simulink model "threePhaseSinePWM"  (R2024b)
settings: Solver=VariableStepAuto  StartTime=0.0  StopTime=5  RelTol=1e-3
libraries: spsMosfetLib x6, spsThreePhaseSeriesRLCBranchLib x2, spsThreePhaseVIMeasurementLib x2, spsDCVoltageSourceLib x1, spsGroundLib x1, spsTriangleGeneratorLib x1, spspowerguiLib x1
settings Model: Creator=lenovo  LastModifiedBy=lenovo

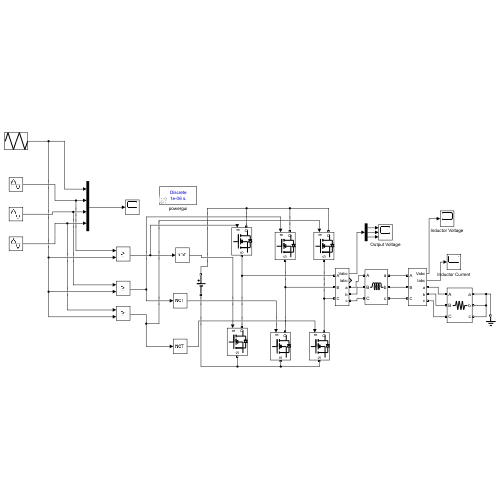
[thumbnail: Simulink's stored preview of the top-level diagram]
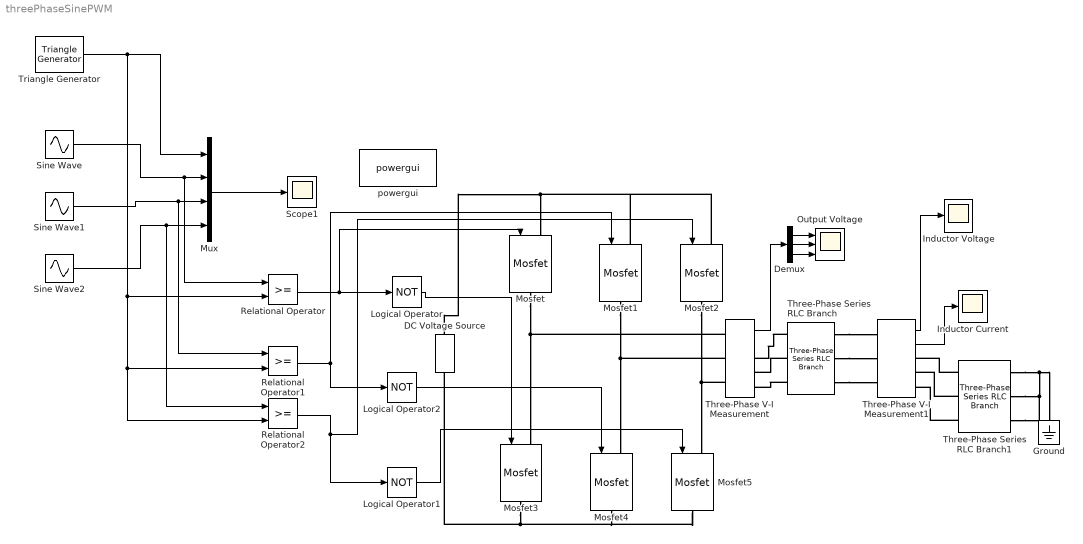
== system threePhaseSinePWM ==
  DC Voltage Source : spsDCVoltageSourceLib/DC Voltage Source  Amplitude=800  Measurements=None
  Demux : Demux  Outputs=3
  Ground : spsGroundLib/Ground  LConnTagsString=a
  Inductor Current : Scope
  Inductor Voltage : Scope
  Logical Operator : Logic  Operator=NOT  AllPortsSameDT=off  OutDataTypeStr=boolean
  Logical Operator1 : Logic  Operator=NOT  AllPortsSameDT=off  OutDataTypeStr=boolean
  Logical Operator2 : Logic  Operator=NOT  AllPortsSameDT=off  OutDataTypeStr=boolean
  Mosfet{,1..5} (6 alike) : spsMosfetLib/Mosfet  Ron=0.1  Lon=0  Rd=0.01  Vfd=0  IC=0  Rs=1e5  Cs=inf  Measurements=off
  Mux : Mux
  Output Voltage : Scope  NumInputPorts=3
  Relational Operator : RelationalOperator  OutDataTypeStr=boolean  RndMeth=Simplest  InputSameDT=off
  Relational Operator1 : RelationalOperator  OutDataTypeStr=boolean  RndMeth=Simplest  InputSameDT=off
  Relational Operator2 : RelationalOperator  OutDataTypeStr=boolean  RndMeth=Simplest  InputSameDT=off
  Scope1 : Scope
  Sine Wave : Sin  Amplitude=0.8  Frequency=2*pi*50  SampleTime=0
  Sine Wave1 : Sin  Amplitude=0.8  Frequency=2*pi*50  Phase=2*pi*50/3  SampleTime=0
  Sine Wave2 : Sin  Amplitude=0.8  Frequency=2*pi*50  Phase=-2*pi*50/3  SampleTime=0
  Three-Phase Series RLC Branch : spsThreePhaseSeriesRLCBranchLib/Three-Phase Series RLC Branch  LConnTagsString=A|B|C  RConnTagsString=A|B|C  BranchType=L  Resistance=1  Inductance=9e-3  Capacitance=1e-6  Measurements=None
  Three-Phase Series RLC Branch1 : spsThreePhaseSeriesRLCBranchLib/Three-Phase Series RLC Branch  LConnTagsString=A|B|C  RConnTagsString=A|B|C  BranchType=R  Resistance=5  Inductance=1e-3  Capacitance=1e-6  Measurements=None
  Three-Phase V-I Measurement : spsThreePhaseVIMeasurementLib/Three-Phase V-I Measurement  VoltageMeasurement=phase-to-ground  SetLabelV=off  LabelV=Vabc  Vpu=off  VpuLL=off  CurrentMeasurement=yes  SetLabelI=off  LabelI=Iabc  Ipu=off  Pbase=100e6  Vbase=500e3  OutputType=Complex  PhasorSimulation=off  PSBequivalent=0
  Three-Phase V-I Measurement1 : spsThreePhaseVIMeasurementLib/Three-Phase V-I Measurement  VoltageMeasurement=phase-to-ground  SetLabelV=off  LabelV=VabcL  Vpu=off  VpuLL=off  CurrentMeasurement=yes  SetLabelI=off  LabelI=IabcL  Ipu=off  Pbase=100e6  Vbase=500e3  OutputType=Complex  PhasorSimulation=off  PSBequivalent=0
  Triangle Generator : spsTriangleGeneratorLib/Triangle Generator  Freq=10e3  Phase=90  Ts=0
  powergui : spspowerguiLib/powergui  Priority=1  SimulationMode=Discrete  SampleTime=1e-6  frequency=60  Iterations=50  frequencyindice=0  Pbase=100e6  ErrMax=1e-4  UnitsV=kV  UnitsW=MW  buscounter=0  FunctionMessages=off  echomessages=off  EnableUseOfTLC=off  CurrentSourceSwitches=off  DisableSnubberDevices=off  DisableRonSwitches=off  DisableVfSwitches=off  DisplayEquations=off  AutomaticDiscreteSolvers=off  SolverType=Tustin/Backward Euler (TBE)  Interpol=off  ExternalGateDelay=off  methode=off  Ts=100  x0status=blocks  SPID=on  SwTol=0  HookPort=off  NonlinearTolerance=1e-4  nMaxIteration=100  ContinueOnMaxIteration=off  RestoreLinks=warning  ResistiveCurrentMeasurement=off  Frange=[0:2:500]  Ylog=off  Xlog=on  ShowGrid=off  save=off  variable=ZData  structure=0  ZoomFFT=off  StartTime=0.0  cycles=1  DisplayStyle=1  fundamental=60  FreqAxis=off  MaxFrequency=1000  frequencyindicesteady=1  RmsSteady=1  display=off
  wires:
  Mux/1 -> Scope1/1
  Sine Wave2/1 -> Mux/4, Relational Operator2/1
  Sine Wave1/1 -> Mux/3, Relational Operator1/1
  Sine Wave/1 -> Mux/2, Relational Operator/1
  Triangle Generator/1 -> Mux/1, Relational Operator2/2, Relational Operator1/2, Relational Operator/2
  Relational Operator/1 -> Mosfet/1, Logical Operator/1
  Logical Operator1/1 -> Mosfet5/1
  Logical Operator2/1 -> Mosfet4/1
  Logical Operator/1 -> Mosfet3/1
  Relational Operator1/1 -> Mosfet1/1, Logical Operator2/1
  Relational Operator2/1 -> Mosfet2/1, Logical Operator1/1
  Three-Phase V-I Measurement1/1 -> Inductor Voltage/1
  Three-Phase V-I Measurement1/2 -> Inductor Current/1
  Demux/3 -> Output Voltage/3
  Demux/1 -> Output Voltage/1
  Demux/2 -> Output Voltage/2
  Three-Phase V-I Measurement/1 -> Demux/1
  connections:
  Mosfet/RConn1 -- Mosfet3/LConn1 -- Three-Phase V-I Measurement/LConn1
  Mosfet1/RConn1 -- Mosfet4/LConn1 -- Three-Phase V-I Measurement/LConn2
  Mosfet2/RConn1 -- Mosfet5/LConn1 -- Three-Phase V-I Measurement/LConn3
  DC Voltage Source/RConn1 -- Mosfet2/LConn1 -- Mosfet1/LConn1 -- Mosfet/LConn1
  Mosfet3/RConn1 -- Mosfet5/RConn1 -- Mosfet4/RConn1 -- DC Voltage Source/LConn1
  Three-Phase Series RLC Branch/LConn1 -- Three-Phase V-I Measurement/RConn1
  Three-Phase Series RLC Branch/LConn2 -- Three-Phase V-I Measurement/RConn2
  Three-Phase Series RLC Branch/LConn3 -- Three-Phase V-I Measurement/RConn3
  Three-Phase Series RLC Branch/RConn1 -- Three-Phase V-I Measurement1/LConn1
  Three-Phase Series RLC Branch/RConn2 -- Three-Phase V-I Measurement1/LConn2
  Three-Phase Series RLC Branch/RConn3 -- Three-Phase V-I Measurement1/LConn3
  Three-Phase Series RLC Branch1/LConn1 -- Three-Phase V-I Measurement1/RConn1
  Three-Phase Series RLC Branch1/LConn2 -- Three-Phase V-I Measurement1/RConn2
  Three-Phase Series RLC Branch1/LConn3 -- Three-Phase V-I Measurement1/RConn3
  Three-Phase Series RLC Branch1/RConn1 -- Three-Phase Series RLC Branch1/RConn3 -- Three-Phase Series RLC Branch1/RConn2 -- Ground/LConn1
